simulink model "Y3Tiltrotor_sim3_IINDI_case2_1"  (R2025a)
settings: Solver=ode4  StartTime=0.0  StopTime=80  FixedStep=uavParam.sampleTime  RelTol=1e-3
PreLoadFcn:
  | filepath  = fileparts(get_param(bdroot, 'FileName'))
  | cd(filepath);
InitFcn:
  | Init_sim_IINDI_case2_1;
values from neighbouring files (symbols this model uses):
  a_HOD_p = 5    [Init_sim_IINDI_case2.m]    (also in Init_sim_IINDI_case2_1.m)
  a_HOD_q = 5    [Init_sim_IINDI_case2.m]    (also in Init_sim_IINDI_case2_1.m = 25)
  a_HOD_r = 5    [Init_sim_IINDI_case2.m]    (also in Init_sim_IINDI_case2_1.m)
  a_HOD_u = 5    [Init_sim_IINDI_case2.m]    (also in Init_sim_IINDI_case2_1.m = 15)
  a_HOD_v = 2    [Init_sim_IINDI_case2.m]    (also in Init_sim_IINDI_case2_1.m)
  a_HOD_w = 30    [Init_sim_IINDI_case2.m]    (also in Init_sim_IINDI_case2_1.m = 10)
  control = struct    [Init_sim_IINDI_case2.m]    (also in Init_sim_IINDI_case2_1.m)
  env = struct    [InitData.m]
  flightState = struct    [Init_sim_IINDI_case2.m]    (also in Init_sim_IINDI_case2_1.m)
  FWSpeed0 = 15    [Init_sim_IINDI_case2.m]    (also in Init_sim_IINDI_case2_1.m)
  k_lpf_p = 50    [Init_sim_IINDI_case2.m]    (also in Init_sim_IINDI_case2_1.m)
  k_lpf_q = 80    [Init_sim_IINDI_case2.m]    (also in Init_sim_IINDI_case2_1.m = 150)
  k_lpf_r = 100    [Init_sim_IINDI_case2.m]    (also in Init_sim_IINDI_case2_1.m)
  k_lpf_u = 8    [Init_sim_IINDI_case2.m]    (also in Init_sim_IINDI_case2_1.m)
  k_lpf_v = 1.5    [Init_sim_IINDI_case2.m]    (also in Init_sim_IINDI_case2_1.m)
  k_lpf_w = 50    [Init_sim_IINDI_case2.m]    (also in Init_sim_IINDI_case2_1.m)
  k_p = 5    [Init_sim_IINDI_case2.m]    (also in Init_sim_IINDI_case2_1.m)
  k_q = 12    [Init_sim_IINDI_case2.m]    (also in Init_sim_IINDI_case2_1.m)
  k_r = 0.1    [Init_sim_IINDI_case2.m]    (also in Init_sim_IINDI_case2_1.m)
  k_u = 0.2    [Init_sim_IINDI_case2.m]    (also in Init_sim_IINDI_case2_1.m = 1)
  k_v = 0.7    [Init_sim_IINDI_case2.m]    (also in Init_sim_IINDI_case2_1.m = 0.2)
  k_w = 2    [Init_sim_IINDI_case2.m]    (also in Init_sim_IINDI_case2_1.m)
  l_p = 30    [Init_sim_IINDI_case2.m]    (also in Init_sim_IINDI_case2_1.m)
  l_q = 15    [Init_sim_IINDI_case2.m]    (also in Init_sim_IINDI_case2_1.m)
  l_r = 25    [Init_sim_IINDI_case2.m]    (also in Init_sim_IINDI_case2_1.m)
  l_u = 1    [Init_sim_IINDI_case2.m]    (also in Init_sim_IINDI_case2_1.m = 0.8)
  l_v = 1.2    [Init_sim_IINDI_case2.m]    (also in Init_sim_IINDI_case2_1.m)
  l_w = 1    [Init_sim_IINDI_case2.m]    (also in Init_sim_IINDI_case2_1.m)
  lamda_p = 10    [Init_sim_IINDI_case2.m]    (also in Init_sim_IINDI_case2_1.m)
  lamda_q = 5    [Init_sim_IINDI_case2.m]    (also in Init_sim_IINDI_case2_1.m)
  lamda_r = 1    [Init_sim_IINDI_case2.m]    (also in Init_sim_IINDI_case2_1.m)
  lamda_u = 1    [Init_sim_IINDI_case2.m]    (also in Init_sim_IINDI_case2_1.m)
  lamda_v = 0.15    [Init_sim_IINDI_case2.m]    (also in Init_sim_IINDI_case2_1.m)
  lamda_w = 1    [Init_sim_IINDI_case2.m]    (also in Init_sim_IINDI_case2_1.m)
  uavParam = struct    [InitData.m]
undefined symbols (not defined in the file or in its folder): a_HOD, a_HOD_uvw, ControlSampleTime, F, Light, MIL, Newton, Raphson
libraries: slpidlib x31, SignalEditorBlockLib x15, simulink x3, aerolibtransform2 x3, sharedtransform x3, robotcorelib x3, matrix_library x3, aerolibasang x2, aerolibutil x2, aerolibwind2 x2, shared6dof x1, aerolibatmos2 x1
(part 8 of 8)

== matlab function Y3Tiltrotor_sim3_IINDI_case2_1/Subsystem/混控器/多旋翼混控/旋翼模态混控/Multirotor Mixer2 传统混控简化版 ==
  data: u_z input; u_phi input; u_theta input; u_psi input; w1 output; w2 output; w3 output; Tilt1 output; Tilt2 output
function [w1,w2,w3,Tilt1,Tilt2] = fcn(u_z,u_phi,u_theta,u_psi)
    
    m = 0.585;
    g = 9.80665;
    rho = 1.225;
    R = 0.765;
    k_1 = 19741.896106*2*pi/60;

    CT = 9.5883e-7;
    CQ = 1.4797e-8;
    R = 0.765;
    l1 = 0.13;
    l2 = 0.24;

    % u_z_bar = u_z - m*g*cos(roll)*cos(pitch)/(CT*rho*pi*R^4*k_1^2);
    u_z_bar = u_z;

    k = (CQ*R)/CT;

    G = [ 1  1   1   0  0;
         -l1 l1  0   0  0;
         l1  l1 -l2  0  0;
         -k   k  0  -l1 l1];
    G_inv = pinv(G);

    u = [u_z_bar,u_phi,u_theta,u_psi]';
    u_act = G_inv*u;

    if u_act(1) < 0
        w1 = 0;
    else
        w1 = u_act(1);
    end

    if u_act(2) < 0
        w2 = 0;
    else
        w2 = u_act(2);
    end

    if u_act(3) < 0
        w3 = 0;
    else
        w3 = u_act(3);
    end
    
    if w1 == 0
        Tilt1 = 0;
    else
        Tilt1 = u_act(4)/w1;
    end

    if w2 == 0
        Tilt2 = 0;
    else
        Tilt2 = u_act(5)/w2;
    end


end

== matlab function Y3Tiltrotor_sim3_IINDI_case2_1/Y3 Tiltrotor Aircraft Model/States Bus/MATLAB Function1 ==
  data: vxyz input; course output; gndSpeed output
function [course, gndSpeed] = fcn(vxyz)

vx = vxyz(1);
vy = vxyz(2);
course = atan2(vy, vx);
gndSpeed = norm([vx vy 0]);

== matlab function Y3Tiltrotor_sim3_IINDI_case2_1/Y3 Tiltrotor Aircraft Model/Subsystem/Aerodynamic Forces and Moments/Compute Body Frame Aerodynamic Forces and Moments/Wind frame F& M/Longitudinal Channel/CD/CD(alpha) ==
  data: alpha input; CD_alpha output
function CD_alpha = piecewise_CD_alpha(alpha)

    c1 = 10.5;
    c2 = 0.023013;
    c3 = 0.000398;
    c4 = 1.077953;
    c5 = -1.061505;
    c6 = 0.919668;
    c7 = -7.769775;
    c8 = 49.988;
    c9 = -0.043323;
    c10 = 1.088698;
    c11 = 0.891002;
    c12 = -9.586878;

    CD_alpha = zeros(size(alpha));

    idx_pos = alpha >= 0;
    if any(idx_pos)
        alpha_pos = alpha(idx_pos);
        CD_alpha(idx_pos) = (1+tanh(c1*(18.4^2-alpha_pos.^2)))/(1+tanh(c1*18.4^2)).*(c2+c3*alpha_pos.^2)...
            +(1-(1+tanh(c1*(18.4^2-alpha_pos.^2)))/(1+tanh(c1*18.4^2))).*(c4+c5*sin(c6*pi/180*alpha_pos+c7).^2);
    end
    
    idx_neg = alpha < 0;
    if any(idx_neg)
        alpha_neg = alpha(idx_neg);
        CD_alpha(idx_neg) = (1+tanh(c8*(15^2-alpha_neg.^2)))/(1+tanh(c8*15^2)).*(c2+c3*alpha_neg.^2)...
            +(1-(1+tanh(c8*(15^2-alpha_neg.^2)))/(1+tanh(c8*15^2))).*(c9+c10*sin(c11*pi/180*alpha_neg+c12).^2);
    end

end

== matlab function Y3Tiltrotor_sim3_IINDI_case2_1/Y3 Tiltrotor Aircraft Model/Subsystem/Aerodynamic Forces and Moments/Compute Body Frame Aerodynamic Forces and Moments/Wind frame F& M/Longitudinal Channel/Cm/Cm(alpha) ==
  data: Cm_alpha output; alpha input
function Cm_alpha = piecewise_Cm_alpha(alpha)

    c1 = 0.000219;
    c2 = -0.011442;
    c3 = 0.056866;
    c4 = -3.422369;
    c5 = -1.763366;
    c6 = -0.059447;
    c7 = 3.052526;
    c8 = 0.000256;
    c9 = -3.005585;
    c10 = -0.035985;
    c11 = -15.643618;

    Cm_alpha = zeros(size(alpha));

    idx_pos = alpha >= 0;
    if any(idx_pos)
        alpha_pos = alpha(idx_pos);
        Cm_alpha(idx_pos) = (1+tanh(c1*(18.4^2-alpha_pos.^2)))/(1+tanh(c1*18.4^2)).*(c2+c3*sin(c4*pi/180*alpha_pos))...
            +(1-(1+tanh(c1*(18.4^2-alpha_pos.^2)))/(1+tanh(c1*18.4^2))).*(c5*sin(c6*pi/180*alpha_pos+c7));
    end
    
    idx_neg = alpha < 0;
    if any(idx_neg)
        alpha_neg = alpha(idx_neg);
        Cm_alpha(idx_neg) = (1+tanh(c8*(15^2-alpha_neg.^2)))/(1+tanh(c8*15^2)).*(c2+c3*sin(c4*pi/180*alpha_neg))...
            +(1-(1+tanh(c8*(15^2-alpha_neg.^2)))/(1+tanh(c8*15^2))).*(c9*sin(c10*pi/180*alpha_neg+c11));
    end

end

== matlab function Y3Tiltrotor_sim3_IINDI_case2_1/Y3 Tiltrotor Aircraft Model/Subsystem/Aerodynamic Forces and Moments/Compute Body Frame Aerodynamic Forces and Moments/Wind frame F& M/Lateral Channel/CY/CY(beta) ==
  data: CY_beta output; beta input
function CY_beta = fcn_CY_beta(beta)

    c1 = 65.424349;
    c2 = 41.5;
    c3 = 0.100430;
    c4 = -1.744107;
    c5 = 0.083409;
    c6 = 1.914772;
    c7 = -3.141796;

    CY_beta = (1+tanh(c1*(c2^2-beta.^2)))/(1+tanh(c1*c2^2)).*(c3*sin(c4*pi/180*beta))...
        + (1-(1+tanh(c1*(c2^2-beta.^2)))/(1+tanh(c1*c2^2))).*(c5*sin(c6*pi/180*beta+c7));

end

== matlab function Y3Tiltrotor_sim3_IINDI_case2_1/Y3 Tiltrotor Aircraft Model/Subsystem/Aerodynamic Forces and Moments/Compute Body Frame Aerodynamic Forces and Moments/Wind frame F& M/Lateral Channel/Cl/Cl(beta) ==
  data: Cl1_beta output; beta input
function Cl1_beta = fcn_Cl1_beta(beta)

    c1 = 18.339628;
    c2 = 41.5;
    c3 = 0.035354;
    c4 = -1.788085;
    c5 = 0.035299;
    c6 = -1.515415;
    c7 = 0.001573;

    Cl1_beta = (1+tanh(c1*(c2^2-beta.^2)))/(1+tanh(c1*c2^2)).*(c3*sin(c4*pi/180*beta))...
        + (1-(1+tanh(c1*(c2^2-beta.^2)))/(1+tanh(c1*c2^2))).*(c5*sin(c6*pi/180*beta+c7));

end

== matlab function Y3Tiltrotor_sim3_IINDI_case2_1/Y3 Tiltrotor Aircraft Model/Subsystem/Aerodynamic Forces and Moments/Compute Body Frame Aerodynamic Forces and Moments/Wind frame F& M/Lateral Channel/Cn/Cn(beta) ==
  data: Cn_beta output; beta input
function Cn_beta = fcn_Cn_beta(beta)

    c1 = 16.018126;
    c2 = 41.5;
    c3 = 0.045296;
    c4 = 0.918923;
    c5 = 0.028417;
    c6 = 1.203453;
    c7 = 6.274968;

    Cn_beta = (1+tanh(c1*(c2^2-beta.^2)))/(1+tanh(c1*c2^2)).*(c3*sin(c4*pi/180*beta))...
        + (1-(1+tanh(c1*(c2^2-beta.^2)))/(1+tanh(c1*c2^2))).*(c5*sin(c6*pi/180*beta+c7));

end

== matlab function Y3Tiltrotor_sim3_IINDI_case2_1/Y3 Tiltrotor Aircraft Model/Subsystem/Aerodynamic Forces and Moments/Compute Body Frame Aerodynamic Forces and Moments/Wind frame F& M/Longitudinal Channel/Cm/Cm(delta_e) ==
  data: delta_e input; Cm_delta_e output
function Cm_delta_e = fcn_Cm_delta_e(delta_e)

    c1 = 0.000301;
    c2 = -1.724970;
    c3 = 0.142608;
    c4 = 0.109046;
    c5 = 0.694663;
    c6 = -2.968985;

    Cm_delta_e = (1+tanh(c1*(47.5^2-delta_e.^2)))/(1+tanh(c1*47.5^2)).*(c2*sin(c3*pi/180*delta_e))...
            +(1-(1+tanh(c1*(47.5^2-delta_e.^2)))/(1+tanh(c1*47.5^2))).*(c4*sin(c5*pi/180*delta_e+c6));

end

== matlab function Y3Tiltrotor_sim3_IINDI_case2_1/Y3 Tiltrotor Aircraft Model/Subsystem/Aerodynamic Forces and Moments/Compute Body Frame Aerodynamic Forces and Moments/Wind frame F& M/Longitudinal Channel/CD/CD(delta_e) ==
  data: delta_e input; CD_delta_e output
function CD_delta_e = fcn_CD_delta_e(delta_e)

    c1 = 0.000707;
    c2 = 0.000057;
    c3 = 0.013601;
    c4 = 0.101850;
    c5 = 1.443831;
    c6 = 56.012704;
    c7 = 0.000024;
    c8 = 0.101300;
    c9 = -0.021731;
    c10 = -3.024408;
    c11 = 61.266062;

    CD_delta_e = zeros(size(delta_e));

    idx_pos = delta_e >= 0;
    if any(idx_pos)
        delta_e_pos = delta_e(idx_pos);
        CD_delta_e(idx_pos) = (1+tanh(c1*(47.4^2-delta_e_pos.^2)))/(1+tanh(c1*47.4^2)).*(c2*delta_e_pos.^2)...
            +(1-(1+tanh(c1*(47.4^2-delta_e_pos.^2)))/(1+tanh(c1*47.4^2))).*(c3+c4*sin(c5*pi/180*delta_e_pos+c6).^2);
    end

    idx_neg = delta_e < 0;
    if any(idx_neg)
        delta_e_neg = delta_e(idx_neg);
        CD_delta_e(idx_neg) = (1+tanh(c1*(47.4^2-delta_e_neg.^2)))/(1+tanh(c1*47.4^2)).*(c7*delta_e_neg.^2)...
            +(1-(1+tanh(c1*(47.4^2-delta_e_neg.^2)))/(1+tanh(c1*47.4^2))).*(c8+c9*sin(c10*pi/180*delta_e_neg+c11).^2);
    end
    
end
